simulink model "PC_Oscilloscope_Simulation"  (R2026a)
settings: Solver=VariableStepAuto  StopTime=1
libraries: simulink x1, eeRmsMeasurement x1
settings Model: Creator=ASUS  LastModifiedBy=ASUS

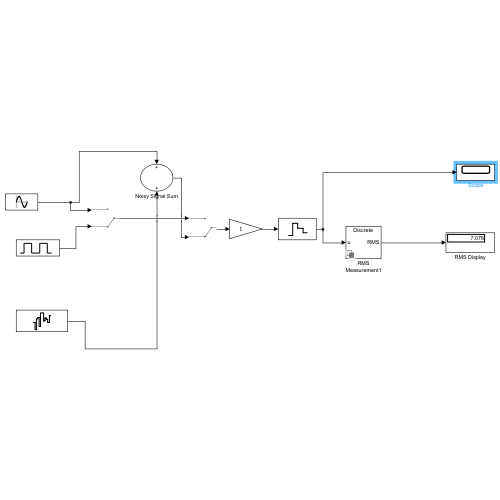
[thumbnail: Simulink's stored preview of the top-level diagram]
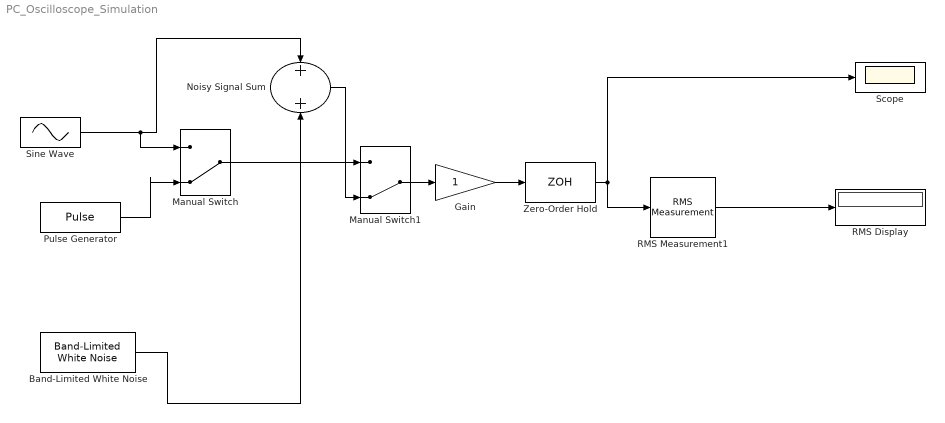
== system PC_Oscilloscope_Simulation ==
  Band-Limited White Noise : simulink/Sources/Band-Limited White Noise  Cov=[0.1]  Ts=0.1  seed=23341
  Gain : Gain
  Manual Switch : ManualSwitch  CurrentSetting=0
  Manual Switch1 : ManualSwitch  CurrentSetting=0
  Noisy Signal Sum : Sum
  Pulse Generator : DiscretePulseGenerator  PulseType=Time based  Amplitude=10  Period=0.02  PulseWidth=50
  RMS Measurement1 : eeRmsMeasurement/RMS Measurement  LabelModeActiveChoice=Total  F=50  SpecifyHarmonics=off  K=[0 1 2]  Ts=0.001
      settings: LibrarySourceBlock=|
      | ee_sl_lib/Measurements/RMS
      | Measurement
  RMS Display : Display
  Scope : Scope
      settings: ActiveDisplayYMinimum=-13.833111861611934  ActiveDisplayYMaximum=15.299969254946273
  Sine Wave : Sin  Amplitude=10  Frequency=314.159  SampleTime=0
  Zero-Order Hold : ZeroOrderHold  SampleTime=0.001
  wires:
  Sine Wave/1 -> Noisy Signal Sum/1, Manual Switch/1
  Pulse Generator/1 -> Manual Switch/2
  Manual Switch/1 -> Manual Switch1/1
  Manual Switch1/1 -> Gain/1
  Gain/1 -> Zero-Order Hold/1
  Zero-Order Hold/1 -> RMS Measurement1/1, Scope/1
  Band-Limited White Noise/1 -> Noisy Signal Sum/2
  Noisy Signal Sum/1 -> Manual Switch1/2
  RMS Measurement1/1 -> RMS Display/1
